simulink model "quadcopter_flight_controller"  (R2026a)
settings: Solver=FixedStepDiscrete  StopTime=10  FixedStep=0.001
settings Model: Creator=sahil  LastModifiedBy=sahil

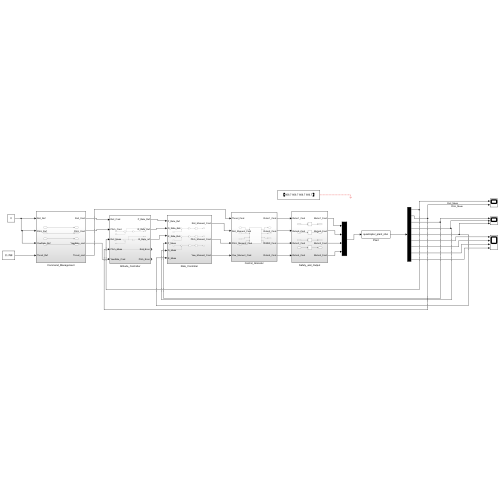
[thumbnail: Simulink's stored preview of the top-level diagram]
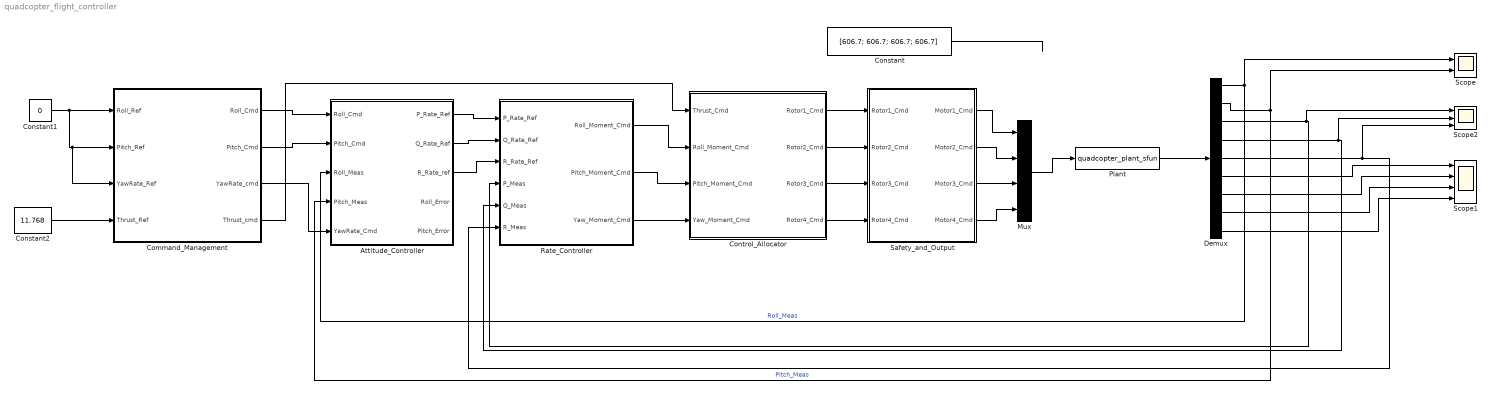
== system quadcopter_flight_controller ==
  Attitude_Controller : Subsystem
  Command_Management : Subsystem
  Constant : Constant  Value=[606.7; 606.7; 606.7; 606.7]  SampleTime=0.001
  Constant1 : Constant  Value=0  SampleTime=0.001
  Constant2 : Constant  Value=11.768  SampleTime=0.001
  Control_Allocator : Subsystem
  Demux : Demux  Outputs=9
  Mux : Mux
  Plant : S-Function  FunctionName=quadcopter_plant_sfun  SFunctionDeploymentMode=off  EnableBusSupport=off
  Rate_Controller : Subsystem
  Safety_and_Output : Subsystem
  Scope : Scope  NumInputPorts=2
      settings: ActiveDisplayYMinimum=-10.269314790379651  ActiveDisplayYMaximum=17.210365217516273
  Scope1 : Scope  NumInputPorts=4
      settings: ActiveDisplayYMinimum=-1  ActiveDisplayYMaximum=1
  Scope2 : Scope  NumInputPorts=3
      settings: ActiveDisplayYMinimum=-1  ActiveDisplayYMaximum=1  DataLoggingVariableName=ScopeData2
  wires:
  Rate_Controller/1(Roll_Moment_Cmd) -> Control_Allocator/2(Roll_Moment_Cmd)
  Attitude_Controller/1(P_Rate_Ref) -> Rate_Controller/1(P_Rate_Ref)
  Command_Management/1(Roll_Cmd) -> Attitude_Controller/1(Roll_Cmd)
  Command_Management/2(Pitch_Cmd) -> Attitude_Controller/2(Pitch_Cmd)
  Attitude_Controller/2(Q_Rate_Ref) -> Rate_Controller/2(Q_Rate_Ref)
  Command_Management/4(Thrust_cmd) -> Control_Allocator/1(Thrust_Cmd)
  Attitude_Controller/3(R_Rate_ref) -> Rate_Controller/3(R_Rate_Ref)
  Rate_Controller/2(Pitch_Moment_Cmd) -> Control_Allocator/3(Pitch_Moment_Cmd)
  Rate_Controller/3(Yaw_Moment_Cmd) -> Control_Allocator/4(Yaw_Moment_Cmd)
  Control_Allocator/1(Rotor1_Cmd) -> Safety_and_Output/1(Rotor1_Cmd)
  Control_Allocator/2(Rotor2_Cmd) -> Safety_and_Output/2(Rotor2_Cmd)
  Control_Allocator/3(Rotor3_Cmd) -> Safety_and_Output/3(Rotor3_Cmd)
  Control_Allocator/4(Rotor4_Cmd) -> Safety_and_Output/4(Rotor4_Cmd)
  Command_Management/3(YawRate_cmd) -> Attitude_Controller/5(YawRate_Cmd)
  Safety_and_Output/1(Motor1_Cmd) -> Mux/1
  Safety_and_Output/2(Motor2_Cmd) -> Mux/2
  Safety_and_Output/3(Motor3_Cmd) -> Mux/3
  Safety_and_Output/4(Motor4_Cmd) -> Mux/4
  Plant/1 -> Demux/1
  Demux/1 -> Attitude_Controller/3(Roll_Meas), Scope/1  "Roll_Meas"
  Demux/2 -> Attitude_Controller/4(Pitch_Meas), Scope/2  "Pitch_Meas"
  Demux/3 -> Scope2/1, Rate_Controller/4(P_Meas)
  Demux/4 -> Scope2/2, Rate_Controller/5(Q_Meas)
  Demux/5 -> Scope2/3, Rate_Controller/6(R_Meas)
  Demux/6 -> Scope1/1
  Demux/7 -> Scope1/2
  Demux/8 -> Scope1/3
  Demux/9 -> Scope1/4
  Constant/1 -> ?
  Mux/1 -> Plant/1
  Constant1/1 -> Command_Management/3(YawRate_Ref), Command_Management/2(Pitch_Ref), Command_Management/1(Roll_Ref)
  Constant2/1 -> Command_Management/4(Thrust_Ref)

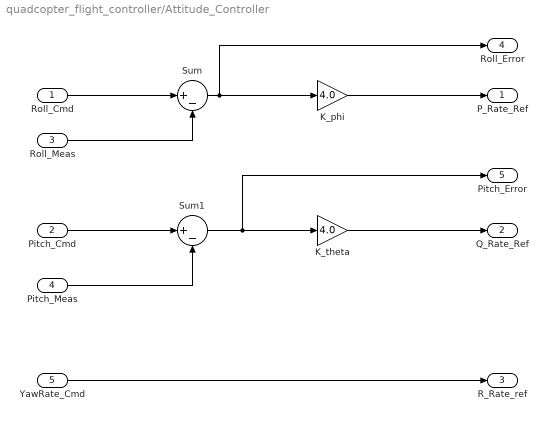
== system quadcopter_flight_controller/Attitude_Controller ==
  Roll_Cmd : Inport
  Pitch_Cmd : Inport  Port=2
  Roll_Meas : Inport  Port=3
  Pitch_Meas : Inport  Port=4
  YawRate_Cmd : Inport  Port=5
  K_phi : Gain  Gain=4.0
  K_theta : Gain  Gain=4.0
  Sum : Sum  Inputs=|+-
  Sum1 : Sum  Inputs=|+-
  P_Rate_Ref : Outport
  Q_Rate_Ref : Outport  Port=2
  R_Rate_ref : Outport  Port=3
  Roll_Error : Outport  Port=4
  Pitch_Error : Outport  Port=5
  wires:
  Roll_Cmd/1 -> Sum/1
  Roll_Meas/1 -> Sum/2
  Sum/1 -> Roll_Error/1, K_phi/1
  K_phi/1 -> P_Rate_Ref/1
  Pitch_Cmd/1 -> Sum1/1
  Pitch_Meas/1 -> Sum1/2
  Sum1/1 -> Pitch_Error/1, K_theta/1
  K_theta/1 -> Q_Rate_Ref/1
  YawRate_Cmd/1 -> R_Rate_ref/1

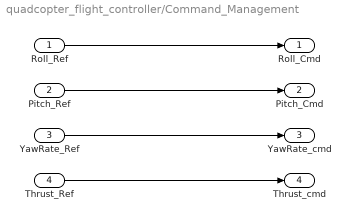
== system quadcopter_flight_controller/Command_Management ==
  Roll_Ref : Inport
  Pitch_Ref : Inport  Port=2
  YawRate_Ref : Inport  Port=3
  Thrust_Ref : Inport  Port=4
  Roll_Cmd : Outport
  Pitch_Cmd : Outport  Port=2
  YawRate_cmd : Outport  Port=3
  Thrust_cmd : Outport  Port=4
  wires:
  Roll_Ref/1 -> Roll_Cmd/1
  Pitch_Ref/1 -> Pitch_Cmd/1
  YawRate_Ref/1 -> YawRate_cmd/1
  Thrust_Ref/1 -> Thrust_cmd/1

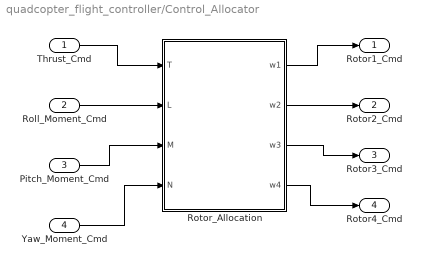
== system quadcopter_flight_controller/Control_Allocator ==
  Thrust_Cmd : Inport
  Roll_Moment_Cmd : Inport  Port=2
  Pitch_Moment_Cmd : Inport  Port=3
  Yaw_Moment_Cmd : Inport  Port=4
  Rotor_Allocation : MATLAB Function  TreatAsAtomicUnit=on
  Rotor1_Cmd : Outport
  Rotor2_Cmd : Outport  Port=2
  Rotor3_Cmd : Outport  Port=3
  Rotor4_Cmd : Outport  Port=4
  wires:
  Thrust_Cmd/1 -> Rotor_Allocation/1(T)
  Roll_Moment_Cmd/1 -> Rotor_Allocation/2(L)
  Pitch_Moment_Cmd/1 -> Rotor_Allocation/3(M)
  Yaw_Moment_Cmd/1 -> Rotor_Allocation/4(N)
  Rotor_Allocation/1(w1) -> Rotor1_Cmd/1
  Rotor_Allocation/2(w2) -> Rotor2_Cmd/1
  Rotor_Allocation/3(w3) -> Rotor3_Cmd/1
  Rotor_Allocation/4(w4) -> Rotor4_Cmd/1

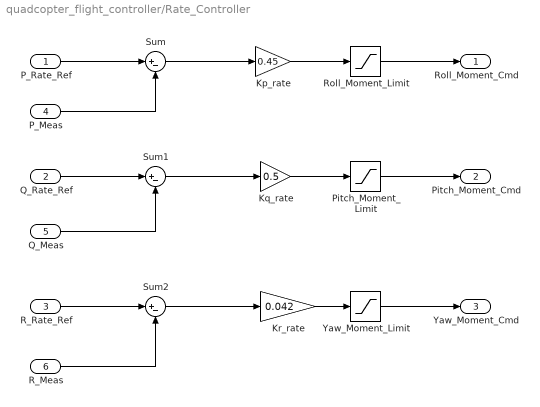
== system quadcopter_flight_controller/Rate_Controller ==
  P_Rate_Ref : Inport
  Q_Rate_Ref : Inport  Port=2
  R_Rate_Ref : Inport  Port=3
  P_Meas : Inport  Port=4
  Q_Meas : Inport  Port=5
  R_Meas : Inport  Port=6
  Kp_rate : Gain  Gain=0.45
  Kq_rate : Gain  Gain=0.5
  Kr_rate : Gain  Gain=0.042
  Pitch_Moment_Limit : Saturate
  Roll_Moment_Limit : Saturate
  Sum : Sum  Inputs=|+-
  Sum1 : Sum  Inputs=|+-
  Sum2 : Sum  Inputs=|+-
  Yaw_Moment_Limit : Saturate  UpperLimit=0.2  LowerLimit=-0.2
  Roll_Moment_Cmd : Outport
  Pitch_Moment_Cmd : Outport  Port=2
  Yaw_Moment_Cmd : Outport  Port=3
  wires:
  P_Meas/1 -> Sum/2
  P_Rate_Ref/1 -> Sum/1
  Sum/1 -> Kp_rate/1
  Kp_rate/1 -> Roll_Moment_Limit/1
  Roll_Moment_Limit/1 -> Roll_Moment_Cmd/1
  Q_Rate_Ref/1 -> Sum1/1
  Q_Meas/1 -> Sum1/2
  Sum1/1 -> Kq_rate/1
  Kq_rate/1 -> Pitch_Moment_Limit/1
  Pitch_Moment_Limit/1 -> Pitch_Moment_Cmd/1
  R_Rate_Ref/1 -> Sum2/1
  R_Meas/1 -> Sum2/2
  Sum2/1 -> Kr_rate/1
  Kr_rate/1 -> Yaw_Moment_Limit/1
  Yaw_Moment_Limit/1 -> Yaw_Moment_Cmd/1

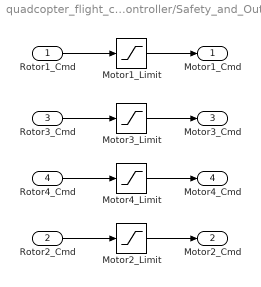
== system quadcopter_flight_controller/Safety_and_Output ==
  Rotor1_Cmd : Inport
  Rotor2_Cmd : Inport  Port=2
  Rotor3_Cmd : Inport  Port=3
  Rotor4_Cmd : Inport  Port=4
  Motor1_Limit : Saturate  UpperLimit=1200  LowerLimit=0
  Motor2_Limit : Saturate  UpperLimit=1200  LowerLimit=0
  Motor3_Limit : Saturate  UpperLimit=1200  LowerLimit=0
  Motor4_Limit : Saturate  UpperLimit=1200  LowerLimit=0
  Motor1_Cmd : Outport
  Motor2_Cmd : Outport  Port=2
  Motor3_Cmd : Outport  Port=3
  Motor4_Cmd : Outport  Port=4
  wires:
  Motor3_Limit/1 -> Motor3_Cmd/1
  Rotor1_Cmd/1 -> Motor1_Limit/1
  Rotor3_Cmd/1 -> Motor3_Limit/1
  Rotor4_Cmd/1 -> Motor4_Limit/1
  Rotor2_Cmd/1 -> Motor2_Limit/1
  Motor1_Limit/1 -> Motor1_Cmd/1
  Motor4_Limit/1 -> Motor4_Cmd/1
  Motor2_Limit/1 -> Motor2_Cmd/1

== matlab function quadcopter_flight_controller/Control_Allocator/Rotor_Allocation ==
  data: T input; w1 output; L input; M input; N input; w2 output; w3 output; w4 output
function [w1, w2, w3, w4] = Rotor_Allocation(T, L, M, N)
%#codegen
% Rotor allocation for a quadcopter.
%
% Inputs:
%   T : Total thrust command [N]
%   L : Roll moment command [N*m]
%   M : Pitch moment command [N*m]
%   N : Yaw moment command [N*m]
%
% Outputs:
%   w1, w2, w3, w4 : Rotor speed commands [rad/s]

% Vehicle and rotor parameters
kT = 8.0e-6;
kQ = 1.5e-7;
d  = 0.141421356;
wMax = 1200.0;

% Control allocation matrix:
% [T; L; M; N] = A * [w1^2; w2^2; w3^2; w4^2]

A = [ kT,    kT,    kT,    kT;
      d*kT, -d*kT, -d*kT,  d*kT;
      d*kT,  d*kT, -d*kT, -d*kT;
      kQ,   -kQ,    kQ,   -kQ ];

% Requested total thrust and moments
wrench = [T; L; M; N];

% Solve for squared rotor speeds
s = A \ wrench;

% Constrain each rotor to its permitted range
s = min(max(s, 0.0), wMax^2);

% Convert squared speed to rotor speed
omega = sqrt(s);

% Individual outputs
w1 = omega(1);
w2 = omega(2);
w3 = omega(3);
w4 = omega(4);
end
